simulink model "ACC_FFNN_trainlm_10_10_10_Nor_Sat_Feb_15_RepFast"  (R2021a)
settings: Solver=FixedStepAuto  StartTime=0.0  StopTime=T  RelTol=1e-3
InitFcn:
  | seed = randi(10000);
StartFcn:
  | seed = randi(10000);
undefined symbols (not defined in the file): amax_ego, amin_ego, patch_sig, safe_patch_sig, sw, t_gap, Ts, v0_ego, v0_lead, v_set, x0_ego, x0_lead, x_gain, x_offset, y_gain, y_offset
libraries: neural x35, simulink x3
(part 2 of 2)

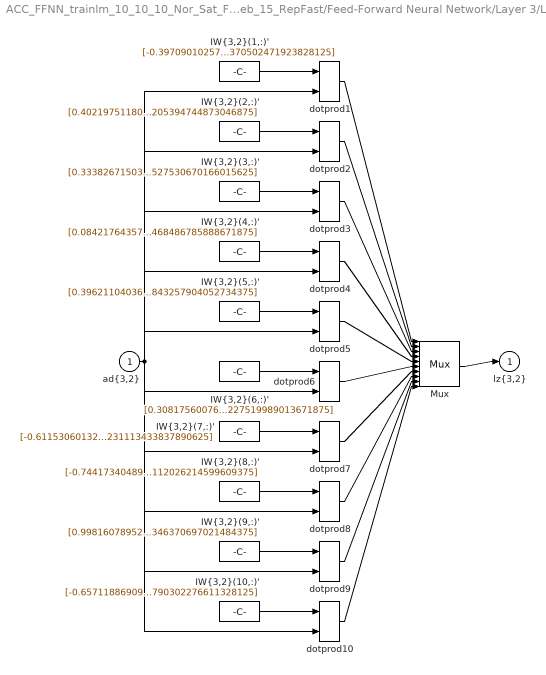
== system ACC_FFNN_trainlm_10_10_10_Nor_Sat_Feb_15_RepFast/Feed-Forward Neural Network/Layer 3/LW{3,2} ==
  "ad{3,2}" : Inport  PortDimensions=10
      mask Display: e = 0.06;c1 = [120 230 180]/255;c2 = ([120 230 180]+0)/(256+128);c3 = ([120 230 180]+128)/(256+128);patch([0 1 1 0],[0 0 1 1],c1);patch([0 1 1 1-e 1-e 0+e],[0 0 1 1-e 0+e 0+e],c2);patch([0 0 1 1-e 0+e 0+e],[0 1 1 1-e 1-e 0+e],c3);plot([0 1 1 0 0],[0 0 1 1 0]);
  "IW{3,2}(1,:)'" : Constant  Value=[-0.39709010257586907499671724508516490459442138671875;-1.0560285868559107225195248247473500669002532958984375;0.20724920121632928182719979304238222539424896240234375;-0.4527379384346807977834714620257727801799774169921875;0.8126163012994658263465908021316863596439361572265625;-0.154315564126900728325608724844641983509063720703125;-0.08013427910105568041654322541944566182792186737060546875;0.2300147839134238647584851378269377164542675018310546875;0.0361042167222083154598522014566697180271148681640625;-0.63583797296403066212633348186500370502471923828125]
      mask Display: e = 0.06;c1 = [120 150 230]/255;c2 = ([120 150 230]+0)/383;c3 = ([120 150 230]+128)/383;patch([0 1 1 0],[0 0 1 1],c1);patch([0 1 1 1-e 1-e 0+e],[0 0 1 1-e 0+e 0+e],c2);patch([0 0 1 1-e 0+e 0+e],[0 1 1 1-e 1-e 0+e],c3);plot([0 1 1 0 0],[0 0 1 1 0]);disp('weights');
  "IW{3,2}(10,:)'" : Constant  Value=[-0.6571188690900326978550083367736078798770904541015625;1.0251229049073398158498093835078179836273193359375;-1.7353656129603944879846721960348077118396759033203125;-2.05008788644529449385345287737436592578887939453125;-0.64246762649526356625528933363966643810272216796875;0.461428191270176590865759180815075524151325225830078125;-1.630466970408159799177383320056833326816558837890625;1.3304060580495071786089056331547908484935760498046875;-0.8640144630599788655445081531070172786712646484375;1.1312937392575890260815185683895833790302276611328125]
      mask Display: e = 0.06;c1 = [120 150 230]/255;c2 = ([120 150 230]+0)/383;c3 = ([120 150 230]+128)/383;patch([0 1 1 0],[0 0 1 1],c1);patch([0 1 1 1-e 1-e 0+e],[0 0 1 1-e 0+e 0+e],c2);patch([0 0 1 1-e 0+e 0+e],[0 1 1 1-e 1-e 0+e],c3);plot([0 1 1 0 0],[0 0 1 1 0]);disp('weights');
  "IW{3,2}(2,:)'" : Constant  Value=[0.40219751180185259187283008941449224948883056640625;0.122399585419320278134591717389412224292755126953125;-0.247455579442336759399267975823022425174713134765625;-0.4191186714460413131888572024763561785221099853515625;0.7593074489638096391530552864423952996730804443359375;-0.81154132222453068123968478175811469554901123046875;0.3088914155141326833842185806133784353733062744140625;-0.153094162074523421068761308561079204082489013671875;0.887245249096775712160933835548348724842071533203125;-0.55191993835156250014506440493278205394744873046875]
      mask Display: e = 0.06;c1 = [120 150 230]/255;c2 = ([120 150 230]+0)/383;c3 = ([120 150 230]+128)/383;patch([0 1 1 0],[0 0 1 1],c1);patch([0 1 1 1-e 1-e 0+e],[0 0 1 1-e 0+e 0+e],c2);patch([0 0 1 1-e 0+e 0+e],[0 1 1 1-e 1-e 0+e],c3);plot([0 1 1 0 0],[0 0 1 1 0]);disp('weights');
  "IW{3,2}(3,:)'" : Constant  Value=[0.333826715033430698742478170970571227371692657470703125;1.1853051530948455205560776448692195117473602294921875;-0.61718891195319269815655616184812970459461212158203125;-0.424304251874145388345738183488720096647739410400390625;0.635521118741283697062272040056996047496795654296875;0.9393303945179349856431372245424427092075347900390625;1.5316485718698575890783786235260777175426483154296875;-1.774172693413309076504447148181498050689697265625;0.27541819614434803753511005197651684284210205078125;-0.1808173505615830178872016631430597044527530670166015625]
      mask Display: e = 0.06;c1 = [120 150 230]/255;c2 = ([120 150 230]+0)/383;c3 = ([120 150 230]+128)/383;patch([0 1 1 0],[0 0 1 1],c1);patch([0 1 1 1-e 1-e 0+e],[0 0 1 1-e 0+e 0+e],c2);patch([0 0 1 1-e 0+e 0+e],[0 1 1 1-e 1-e 0+e],c3);plot([0 1 1 0 0],[0 0 1 1 0]);disp('weights');
  "IW{3,2}(4,:)'" : Constant  Value=[0.0842176435735496886625384149738238193094730377197265625;-0.1635869170295803642911636188728152774274349212646484375;-1.689697025338983582543050943058915436267852783203125;0.004960934987528893037878052751921131857670843601226806640625;-0.4785440018890707580823118405533023178577423095703125;1.189453553135259245010502127115614712238311767578125;-0.13824973572095988760821683172252960503101348876953125;-0.436935158885420726893045184624497778713703155517578125;0.9153878796831664832467367887147702276706695556640625;0.9096662972944187242063662779401056468486785888671875]
      mask Display: e = 0.06;c1 = [120 150 230]/255;c2 = ([120 150 230]+0)/383;c3 = ([120 150 230]+128)/383;patch([0 1 1 0],[0 0 1 1],c1);patch([0 1 1 1-e 1-e 0+e],[0 0 1 1-e 0+e 0+e],c2);patch([0 0 1 1-e 0+e 0+e],[0 1 1 1-e 1-e 0+e],c3);plot([0 1 1 0 0],[0 0 1 1 0]);disp('weights');
  "IW{3,2}(5,:)'" : Constant  Value=[0.396211040360616717492803218192420899868011474609375;-0.6191334656400917513252579738036729395389556884765625;-0.0359558779362874059160049000638537108898162841796875;0.64875253337767002648206471349112689495086669921875;0.1887125013286616859176092475536279380321502685546875;0.39189862660321583831546377041377127170562744140625;0.436717886411767342025314064812846481800079345703125;-0.69268656481738677399562220671214163303375244140625;-0.5185859290396794829547388872015289962291717529296875;-0.3110751773979156808991319849155843257904052734375]
      mask Display: e = 0.06;c1 = [120 150 230]/255;c2 = ([120 150 230]+0)/383;c3 = ([120 150 230]+128)/383;patch([0 1 1 0],[0 0 1 1],c1);patch([0 1 1 1-e 1-e 0+e],[0 0 1 1-e 0+e 0+e],c2);patch([0 0 1 1-e 0+e 0+e],[0 1 1 1-e 1-e 0+e],c3);plot([0 1 1 0 0],[0 0 1 1 0]);disp('weights');
  "IW{3,2}(6,:)'" : Constant  Value=[0.308175600761394274940130344475619494915008544921875;-0.03187485853883269271147327117432723753154277801513671875;-1.1129112085261831932569975833757780492305755615234375;0.60963332631021194263354345821426250040531158447265625;-0.9549748145195364745774213588447310030460357666015625;0.0176563521433867089138747275001151137985289096832275390625;0.91392785553700772727125922756385989487171173095703125;-0.060216297794634936202395891768901492469012737274169921875;0.35224460772750365578076525707729160785675048828125;0.88467580379154753256187859733472578227519989013671875]
      mask Display: e = 0.06;c1 = [120 150 230]/255;c2 = ([120 150 230]+0)/383;c3 = ([120 150 230]+128)/383;patch([0 1 1 0],[0 0 1 1],c1);patch([0 1 1 1-e 1-e 0+e],[0 0 1 1-e 0+e 0+e],c2);patch([0 0 1 1-e 0+e 0+e],[0 1 1 1-e 1-e 0+e],c3);plot([0 1 1 0 0],[0 0 1 1 0]);disp('weights');
  "IW{3,2}(7,:)'" : Constant  Value=[-0.61153060132377934365877081290818750858306884765625;0.09296216089717058983499242685866192914545536041259765625;0.793970818249388088361229165457189083099365234375;0.69975109131576396226392944299732334911823272705078125;-0.1494813595717301435428225886425934731960296630859375;0.515984781937034231447114507318474352359771728515625;0.272282459886035776985835354935261420905590057373046875;-0.5411180895457008421800537689705379307270050048828125;-0.4218708566510465107768368397955782711505889892578125;-0.309060558407142915715581921176635660231113433837890625]
      mask Display: e = 0.06;c1 = [120 150 230]/255;c2 = ([120 150 230]+0)/383;c3 = ([120 150 230]+128)/383;patch([0 1 1 0],[0 0 1 1],c1);patch([0 1 1 1-e 1-e 0+e],[0 0 1 1-e 0+e 0+e],c2);patch([0 0 1 1-e 0+e 0+e],[0 1 1 1-e 1-e 0+e],c3);plot([0 1 1 0 0],[0 0 1 1 0]);disp('weights');
  "IW{3,2}(8,:)'" : Constant  Value=[-0.74417340489373973166919995492207817733287811279296875;1.7812704318613985510211250584688968956470489501953125;-2.0344480262632966827140990062616765499114990234375;-1.1223070254535780776450337725691497325897216796875;-0.3745622263587689015906789791188202798366546630859375;-2.19131383833174187003578481380827724933624267578125;0.8308885771234688633057885454036295413970947265625;0.177563972793616964285234871567809022963047027587890625;0.3436163308284303496975553571246564388275146484375;-1.765314374507482853005058132112026214599609375]
      mask Display: e = 0.06;c1 = [120 150 230]/255;c2 = ([120 150 230]+0)/383;c3 = ([120 150 230]+128)/383;patch([0 1 1 0],[0 0 1 1],c1);patch([0 1 1 1-e 1-e 0+e],[0 0 1 1-e 0+e 0+e],c2);patch([0 0 1 1-e 0+e 0+e],[0 1 1 1-e 1-e 0+e],c3);plot([0 1 1 0 0],[0 0 1 1 0]);disp('weights');
  "IW{3,2}(9,:)'" : Constant  Value=[0.99816078952272135893508675508201122283935546875;-0.6871900955468730476383143468410708010196685791015625;-0.230761751261178371663618236198090016841888427734375;0.1681386665569040150813862055656500160694122314453125;-0.677030511376500054865346100996248424053192138671875;-0.862387801763897510198830786976031959056854248046875;-0.7887415933419561486772408898104913532733917236328125;-0.08515126862465205448415872524492442607879638671875;0.39028099910347435752555611543357372283935546875;0.204340975163590510277344947098754346370697021484375]
      mask Display: e = 0.06;c1 = [120 150 230]/255;c2 = ([120 150 230]+0)/383;c3 = ([120 150 230]+128)/383;patch([0 1 1 0],[0 0 1 1],c1);patch([0 1 1 1-e 1-e 0+e],[0 0 1 1-e 0+e 0+e],c2);patch([0 0 1 1-e 0+e 0+e],[0 1 1 1-e 1-e 0+e],c3);plot([0 1 1 0 0],[0 0 1 1 0]);disp('weights');
  Mux : Mux  Inputs=10
      mask Display: e = 0.06;c1 = [120 150 230]/255;c2 = ([120 150 230]+0)/383;c3 = ([120 150 230]+128)/383;patch([0 1 1 0],[0 0 1 1],c1);patch([0 1 1 1-e 1-e 0+e],[0 0 1 1-e 0+e 0+e],c2);patch([0 0 1 1-e 0+e 0+e],[0 1 1 1-e 1-e 0+e],c3);plot([0 1 1 0 0],[0 0 1 1 0]);disp('Mux');
  dotprod{1..10} (10 alike) : neural/Weight Functions/dotprod
  "lz{3,2}" : Outport
      mask Display: e = 0.06;c1 = [120 230 180]/255;c2 = ([120 230 180]+0)/(256+128);c3 = ([120 230 180]+128)/(256+128);patch([0 1 1 0],[0 0 1 1],c1);patch([0 1 1 1-e 1-e 0+e],[0 0 1 1-e 0+e 0+e],c2);patch([0 0 1 1-e 0+e 0+e],[0 1 1 1-e 1-e 0+e],c3);plot([0 1 1 0 0],[0 0 1 1 0]);
  wires:
  "IW{3,2}(1,:)'"/1 -> dotprod1/1
  "ad{3,2}"/1 -> dotprod1/2, dotprod2/2, dotprod3/2, dotprod4/2, dotprod5/2, dotprod6/2, dotprod7/2, dotprod8/2, dotprod9/2, dotprod10/2
  dotprod1/1 -> Mux/1
  "IW{3,2}(2,:)'"/1 -> dotprod2/1
  dotprod2/1 -> Mux/2
  "IW{3,2}(3,:)'"/1 -> dotprod3/1
  dotprod3/1 -> Mux/3
  "IW{3,2}(4,:)'"/1 -> dotprod4/1
  dotprod4/1 -> Mux/4
  "IW{3,2}(5,:)'"/1 -> dotprod5/1
  dotprod5/1 -> Mux/5
  "IW{3,2}(6,:)'"/1 -> dotprod6/1
  dotprod6/1 -> Mux/6
  "IW{3,2}(7,:)'"/1 -> dotprod7/1
  dotprod7/1 -> Mux/7
  "IW{3,2}(8,:)'"/1 -> dotprod8/1
  dotprod8/1 -> Mux/8
  "IW{3,2}(9,:)'"/1 -> dotprod9/1
  dotprod9/1 -> Mux/9
  "IW{3,2}(10,:)'"/1 -> dotprod10/1
  dotprod10/1 -> Mux/10
  Mux/1 -> "lz{3,2}"/1

== system ACC_FFNN_trainlm_10_10_10_Nor_Sat_Feb_15_RepFast/Feed-Forward Neural Network/Layer 4/Delays 1 ==
  "p{4}" : Inport  PortDimensions=10
      mask Display: e = 0.06;c1 = [120 230 180]/255;c2 = ([120 230 180]+0)/(256+128);c3 = ([120 230 180]+128)/(256+128);patch([0 1 1 0],[0 0 1 1],c1);patch([0 1 1 1-e 1-e 0+e],[0 0 1 1-e 0+e 0+e],c2);patch([0 0 1 1-e 0+e 0+e],[0 1 1 1-e 1-e 0+e],c3);plot([0 1 1 0 0],[0 0 1 1 0]);
  mux : Mux  Inputs=1
      mask Display: e = 0.06;c1 = [120 150 230]/255;c2 = ([120 150 230]+0)/383;c3 = ([120 150 230]+128)/383;patch([0 1 1 0],[0 0 1 1],c1);patch([0 1 1 1-e 1-e 0+e],[0 0 1 1-e 0+e 0+e],c2);patch([0 0 1 1-e 0+e 0+e],[0 1 1 1-e 1-e 0+e],c3);plot([0 1 1 0 0],[0 0 1 1 0]);disp('Mux')
  "pd{4,3}" : Outport
      mask Display: e = 0.06;c1 = [120 230 180]/255;c2 = ([120 230 180]+0)/(256+128);c3 = ([120 230 180]+128)/(256+128);patch([0 1 1 0],[0 0 1 1],c1);patch([0 1 1 1-e 1-e 0+e],[0 0 1 1-e 0+e 0+e],c2);patch([0 0 1 1-e 0+e 0+e],[0 1 1 1-e 1-e 0+e],c3);plot([0 1 1 0 0],[0 0 1 1 0]);
  wires:
  "p{4}"/1 -> mux/1
  mux/1 -> "pd{4,3}"/1

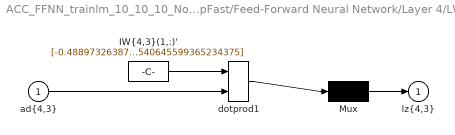
== system ACC_FFNN_trainlm_10_10_10_Nor_Sat_Feb_15_RepFast/Feed-Forward Neural Network/Layer 4/LW{4,3} ==
  "ad{4,3}" : Inport  PortDimensions=10
      mask Display: e = 0.06;c1 = [120 230 180]/255;c2 = ([120 230 180]+0)/(256+128);c3 = ([120 230 180]+128)/(256+128);patch([0 1 1 0],[0 0 1 1],c1);patch([0 1 1 1-e 1-e 0+e],[0 0 1 1-e 0+e 0+e],c2);patch([0 0 1 1-e 0+e 0+e],[0 1 1 1-e 1-e 0+e],c3);plot([0 1 1 0 0],[0 0 1 1 0]);
  "IW{4,3}(1,:)'" : Constant  Value=[-0.488973263878265951287716006845585070550441741943359375;0.443516066782204898544250681879930198192596435546875;-2.5508371281030317589966216473840177059173583984375;-2.0527260793866535237839343608357012271881103515625;-0.3177507859017814073609997649327851831912994384765625;3.731123690264005168977512472139324017916806042194366455078125e-05;-1.0413713158004480607843333928030915558338165283203125;3.739641198398004462433164007961750030517578125;-0.514300803363661795941652599140070378780364990234375;3.533538043299111475192830766900442540645599365234375]
      mask Display: e = 0.06;c1 = [120 150 230]/255;c2 = ([120 150 230]+0)/383;c3 = ([120 150 230]+128)/383;patch([0 1 1 0],[0 0 1 1],c1);patch([0 1 1 1-e 1-e 0+e],[0 0 1 1-e 0+e 0+e],c2);patch([0 0 1 1-e 0+e 0+e],[0 1 1 1-e 1-e 0+e],c3);plot([0 1 1 0 0],[0 0 1 1 0]);disp('weights');
  Mux : Mux  Inputs=1
      mask Display: e = 0.06;c1 = [120 150 230]/255;c2 = ([120 150 230]+0)/383;c3 = ([120 150 230]+128)/383;patch([0 1 1 0],[0 0 1 1],c1);patch([0 1 1 1-e 1-e 0+e],[0 0 1 1-e 0+e 0+e],c2);patch([0 0 1 1-e 0+e 0+e],[0 1 1 1-e 1-e 0+e],c3);plot([0 1 1 0 0],[0 0 1 1 0]);disp('Mux');
  dotprod1 : neural/Weight Functions/dotprod
  "lz{4,3}" : Outport
      mask Display: e = 0.06;c1 = [120 230 180]/255;c2 = ([120 230 180]+0)/(256+128);c3 = ([120 230 180]+128)/(256+128);patch([0 1 1 0],[0 0 1 1],c1);patch([0 1 1 1-e 1-e 0+e],[0 0 1 1-e 0+e 0+e],c2);patch([0 0 1 1-e 0+e 0+e],[0 1 1 1-e 1-e 0+e],c3);plot([0 1 1 0 0],[0 0 1 1 0]);
  wires:
  "IW{4,3}(1,:)'"/1 -> dotprod1/1
  "ad{4,3}"/1 -> dotprod1/2
  dotprod1/1 -> Mux/1
  Mux/1 -> "lz{4,3}"/1
